simulink model "SIXDOF28"  (R2025b)
settings: Solver=VariableStepAuto  StartTime=0.0  StopTime=sortieStopTime_s  MaxStep=2.0  RelTol=1e-3
undefined symbols (not defined in the file): aircraft_mass, alpha0, alpha_bp, b, CL_table, ClCsurfaces, Cldampingrates, Cldeltae, CmCsurfaces, Cmdampingrates, CnCsurfaces, Cndampingrates, COP, CruiseSpeed, deg, density, DiscIntNeverNeededParam, dwGrad, ElTrim, g, h0, InitialHeadingRadBySortie, InitialPosBySortie, InitPitch, InitUb, Initwb, l, lt, maxPropRad, payloadvolume, PitchTrim, rad, rho, s, S, selectedSortie, St, ThrottleTrim
libraries: slpidlib x12, aerolibasang x3, aerolibconvert2 x2, aerolibadyn x1
(part 2 of 3)

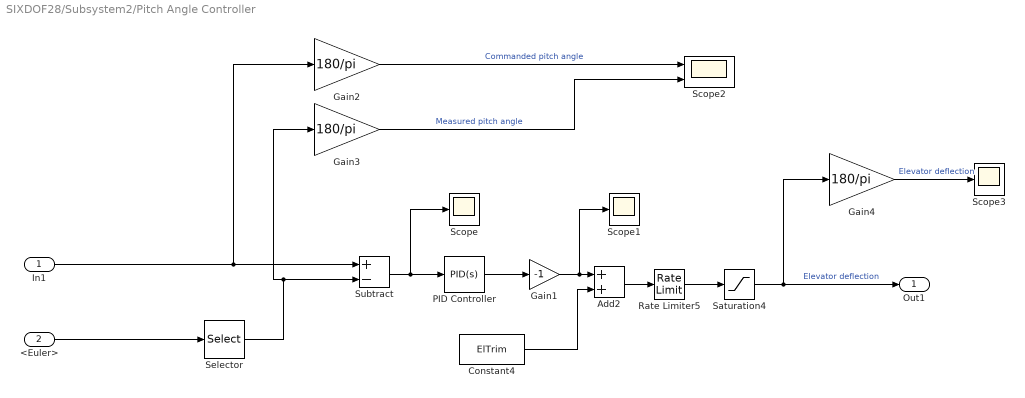
== system SIXDOF28/Subsystem2/Pitch Angle Controller ==
  In1 : Inport
  <Euler> : Inport  Port=2
  Add2 : Sum
  Constant4 : Constant  Value=ElTrim
  Gain1 : Gain  Gain=-1
  Gain2 : Gain  Gain=180/pi
  Gain3 : Gain  Gain=180/pi
  Gain4 : Gain  Gain=180/pi
  PID Controller : slpidlib/PID Controller  Controller=PID  Form=Parallel  TimeDomain=Continuous-time  UseExternalTs=off  SampleTime=-1  IntegratorMethod=Forward Euler  FilterMethod=Forward Euler  ControllerParametersSource=internal  P=1  I=0.2  UseKiTs=off  D=0.1  UseExternalDerivativeSource=off  N=100  UseFilter=on  TunerSelectOption=Transfer Function Based (PID Tuner App)  InitialConditionSource=internal  InitialConditionForIntegrator=0  InitialConditionForFilter=0  DifferentiatorICPrevScaledInput=0  ExternalReset=none  TrackingMode=off  Kt=1  LimitOutput=off  SatLimitsSource=internal  UpperSaturationLimit=inf  LowerSaturationLimit=-inf  LinearizeAsGain=on  AntiWindupMode=none  Kb=1  LimitIntegrator=off  UpperIntegratorSaturationLimit=inf  LowerIntegratorSaturationLimit=-inf  POutMin=[]  POutMax=[]  IOutMin=[]  IOutMax=[]  DOutMin=[]  DOutMax=[]  NOutMin=[]  NOutMax=[]  SumOutMin=[]  SumOutMax=[]  SaturationOutMin=[]  SaturationOutMax=[]  PParamMin=[]  PParamMax=[]  IParamMin=[]  IParamMax=[]  DParamMin=[]  DParamMax=[]  NParamMin=[]  NParamMax=[]  KbParamMin=[]  KbParamMax=[]  KtParamMin=[]  KtParamMax=[]  KbOutMin=[]  KbOutMax=[]  KtOutMin=[]  KtOutMax=[]  IntegratorOutMin=[]  IntegratorOutMax=[]  FilterOutMin=[]  FilterOutMax=[]  SumI1OutMin=[]  SumI1OutMax=[]  SumI2OutMin=[]  SumI2OutMax=[]  SumI3OutMin=[]  SumI3OutMax=[]  SumI4OutMin=[]  SumI4OutMax=[]  SumDOutMin=[]  SumDOutMax=[]  DifferentiatorOutMin=[]  DifferentiatorOutMax=[]  FilterDiffOutCoefMin=[]  FilterDiffOutCoefMax=[]  ReciprocalOutMin=[]  ReciprocalOutMax=[]  SumDenOutMin=[]  SumDenOutMax=[]  SumNumOutMin=[]  SumNumOutMax=[]  DivideOutMin=[]  DivideOutMax=[]  UdiffTsProdOutMin=[]  UdiffTsProdOutMax=[]  NTsProdOutMin=[]  NTsProdOutMax=[]  UintegralTsProdOutMin=[]  UintegralTsProdOutMax=[]  UngainTsProdOutMin=[]  UngainTsProdOutMax=[]  ClampingZeroOutDataTypeStr=Inherit: Inherit via back propagation  ClampingZeroOutMin=[]  ClampingZeroOutMax=[]  FilterDenConstantOutDataTypeStr=Inherit: Inherit via back propagation  FilterDenConstantOutMin=[]  FilterDenConstantOutMax=[]  PCopyOutDataTypeStr=Inherit: Inherit via back propagation  PCopyOutMin=[]  PCopyOutMax=[]  NCopyOutDataTypeStr=Inherit: Inherit via back propagation  NCopyOutMin=[]  NCopyOutMax=[]  IntegratorContinuousStateAttributes=''  IntegratorStateMustResolveToSignalObject=off  IntegratorRTWStateStorageClass=Auto  FilterContinuousStateAttributes=''  FilterStateMustResolveToSignalObject=off  FilterRTWStateStorageClass=Auto  ParallelPVariant=InternalParameters  IdealPVariant=Disabled  IVariant=InternalParameters  DVariant=InternalParameters  IntegratorVariant=Continuous  SatVariant=Disabled  AWVariant=Passthrough  PCopyVariant=Disabled  TRVariant=Disabled  FdbkBlocksVariant=Forward  IdealPFdbkVariant=Disabled  SatFdbkVariant=Disabled  DerivativeFilterVariant=ContFilter  NVariant=InternalParameters  NCopyVariant=Disabled  FilterICVariant=InternalICsFilter  IntegratorICVariant=InternalICs  ExternalResetVariant=Disabled  TRSumVariant=Passthrough  SumFdbkVariant=Disabled  SumVariant=Sum_PID  TsampFilterVariant=InternalTs  TsampNgainVariant=Passthrough  TsampIntegralVariant=Disabled_SignalSpec  ExternalSaturationOutDataTypeStr=Inherit: Same as second input  DerivativeSourceVariant=ErrorSignal  PreIntVariant=InternalPreInt
  Rate Limiter5 : RateLimiter  RisingSlewLimit=1.9  FallingSlewLimit=-1.9
  Saturation4 : Saturate  UpperLimit=21*(pi/180)  LowerLimit=-21*(pi/180)
  Scope : Scope
      settings: ActiveDisplayYMinimum=-1  ActiveDisplayYMaximum=1  DataLoggingVariableName=ScopeData3
  Scope1 : Scope
      settings: ActiveDisplayYMinimum=-1  ActiveDisplayYMaximum=1  DataLoggingVariableName=ScopeData4
  Scope2 : Scope  NumInputPorts=2
      settings: Title=Full Spray mission - Sortie 46  ActiveDisplayYMinimum=-9.9138106361202727  ActiveDisplayYMaximum=18.372173072450739  DataLoggingVariableName=ScopeData56
  Scope3 : Scope
      settings: DataLoggingVariableName=ScopeData81
  Selector : Selector  InputPortWidth=3  IndexOptions=Index vector (dialog)  Indices=[2]  OutputSizes=1
  Subtract : Sum  Inputs=+-
  Out1 : Outport
  wires:
  Gain3/1 -> Scope2/2  "Measured pitch angle"
  Rate Limiter5/1 -> Saturation4/1
  Add2/1 -> Rate Limiter5/1
  Constant4/1 -> Add2/2
  Subtract/1 -> PID Controller/1, Scope/1
  Selector/1 -> Subtract/2, Gain3/1
  In1/1 -> Subtract/1, Gain2/1
  Gain2/1 -> Scope2/1  "Commanded pitch angle"
  PID Controller/1 -> Gain1/1
  <Euler>/1 -> Selector/1
  Gain1/1 -> Scope1/1, Add2/1
  Saturation4/1 -> Gain4/1, Out1/1  "Elevator deflection"
  Gain4/1 -> Scope3/1  "Elevator deflection"

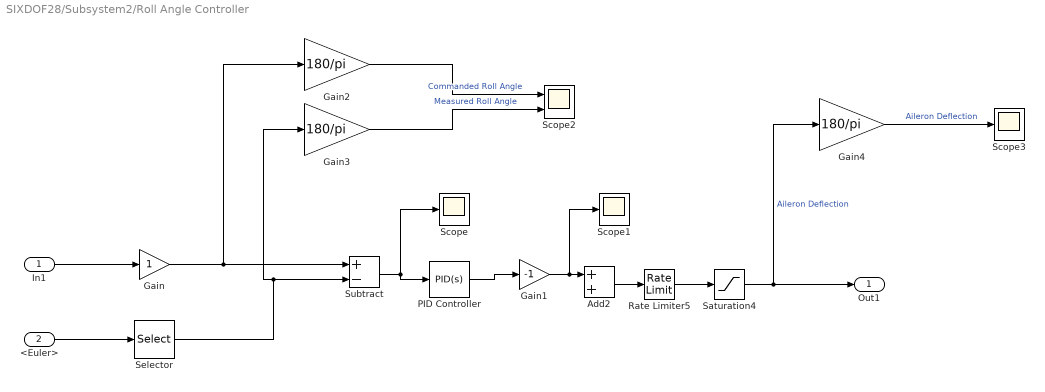
== system SIXDOF28/Subsystem2/Roll Angle Controller ==
  In1 : Inport
  <Euler> : Inport  Port=2
  Add2 : Sum
  Gain : Gain
  Gain1 : Gain  Gain=-1
  Gain2 : Gain  Gain=180/pi
  Gain3 : Gain  Gain=180/pi
  Gain4 : Gain  Gain=180/pi
  PID Controller : slpidlib/PID Controller  Controller=PID  Form=Parallel  TimeDomain=Continuous-time  UseExternalTs=off  SampleTime=-1  IntegratorMethod=Forward Euler  FilterMethod=Forward Euler  ControllerParametersSource=internal  P=5  I=0  UseKiTs=off  D=0  UseExternalDerivativeSource=off  N=100  UseFilter=on  TunerSelectOption=Transfer Function Based (PID Tuner App)  InitialConditionSource=internal  InitialConditionForIntegrator=0  InitialConditionForFilter=0  DifferentiatorICPrevScaledInput=0  ExternalReset=none  TrackingMode=off  Kt=1  LimitOutput=off  SatLimitsSource=internal  UpperSaturationLimit=inf  LowerSaturationLimit=-inf  LinearizeAsGain=on  AntiWindupMode=none  Kb=1  LimitIntegrator=off  UpperIntegratorSaturationLimit=inf  LowerIntegratorSaturationLimit=-inf  POutMin=[]  POutMax=[]  IOutMin=[]  IOutMax=[]  DOutMin=[]  DOutMax=[]  NOutMin=[]  NOutMax=[]  SumOutMin=[]  SumOutMax=[]  SaturationOutMin=[]  SaturationOutMax=[]  PParamMin=[]  PParamMax=[]  IParamMin=[]  IParamMax=[]  DParamMin=[]  DParamMax=[]  NParamMin=[]  NParamMax=[]  KbParamMin=[]  KbParamMax=[]  KtParamMin=[]  KtParamMax=[]  KbOutMin=[]  KbOutMax=[]  KtOutMin=[]  KtOutMax=[]  IntegratorOutMin=[]  IntegratorOutMax=[]  FilterOutMin=[]  FilterOutMax=[]  SumI1OutMin=[]  SumI1OutMax=[]  SumI2OutMin=[]  SumI2OutMax=[]  SumI3OutMin=[]  SumI3OutMax=[]  SumI4OutMin=[]  SumI4OutMax=[]  SumDOutMin=[]  SumDOutMax=[]  DifferentiatorOutMin=[]  DifferentiatorOutMax=[]  FilterDiffOutCoefMin=[]  FilterDiffOutCoefMax=[]  ReciprocalOutMin=[]  ReciprocalOutMax=[]  SumDenOutMin=[]  SumDenOutMax=[]  SumNumOutMin=[]  SumNumOutMax=[]  DivideOutMin=[]  DivideOutMax=[]  UdiffTsProdOutMin=[]  UdiffTsProdOutMax=[]  NTsProdOutMin=[]  NTsProdOutMax=[]  UintegralTsProdOutMin=[]  UintegralTsProdOutMax=[]  UngainTsProdOutMin=[]  UngainTsProdOutMax=[]  ClampingZeroOutDataTypeStr=Inherit: Inherit via back propagation  ClampingZeroOutMin=[]  ClampingZeroOutMax=[]  FilterDenConstantOutDataTypeStr=Inherit: Inherit via back propagation  FilterDenConstantOutMin=[]  FilterDenConstantOutMax=[]  PCopyOutDataTypeStr=Inherit: Inherit via back propagation  PCopyOutMin=[]  PCopyOutMax=[]  NCopyOutDataTypeStr=Inherit: Inherit via back propagation  NCopyOutMin=[]  NCopyOutMax=[]  IntegratorContinuousStateAttributes=''  IntegratorStateMustResolveToSignalObject=off  IntegratorRTWStateStorageClass=Auto  FilterContinuousStateAttributes=''  FilterStateMustResolveToSignalObject=off  FilterRTWStateStorageClass=Auto  ParallelPVariant=InternalParameters  IdealPVariant=Disabled  IVariant=InternalParameters  DVariant=InternalParameters  IntegratorVariant=Continuous  SatVariant=Disabled  AWVariant=Passthrough  PCopyVariant=Disabled  TRVariant=Disabled  FdbkBlocksVariant=Forward  IdealPFdbkVariant=Disabled  SatFdbkVariant=Disabled  DerivativeFilterVariant=ContFilter  NVariant=InternalParameters  NCopyVariant=Disabled  FilterICVariant=InternalICsFilter  IntegratorICVariant=InternalICs  ExternalResetVariant=Disabled  TRSumVariant=Passthrough  SumFdbkVariant=Disabled  SumVariant=Sum_PID  TsampFilterVariant=InternalTs  TsampNgainVariant=Passthrough  TsampIntegralVariant=Disabled_SignalSpec  ExternalSaturationOutDataTypeStr=Inherit: Same as second input  DerivativeSourceVariant=ErrorSignal  PreIntVariant=InternalPreInt
  Rate Limiter5 : RateLimiter  RisingSlewLimit=2.6  FallingSlewLimit=-2.6  SampleTimeMode=inherited
  Saturation4 : Saturate  UpperLimit=14*(pi/180)  LowerLimit=-14*(pi/180)
  Scope : Scope
      settings: ActiveDisplayYMinimum=-1  ActiveDisplayYMaximum=1  DataLoggingVariableName=ScopeData3
  Scope1 : Scope
      settings: ActiveDisplayYMinimum=-1  ActiveDisplayYMaximum=1  DataLoggingVariableName=ScopeData4
  Scope2 : Scope  NumInputPorts=2
      settings: ActiveDisplayYMinimum=-42.530693080397832  ActiveDisplayYMaximum=41.118768188117421  DataLoggingVariableName=ScopeData56
  Scope3 : Scope
      settings: ActiveDisplayYMinimum=-17.5  ActiveDisplayYMaximum=17.5  DataLoggingVariableName=ScopeData70
  Selector : Selector  InputPortWidth=3  IndexOptions=Index vector (dialog)  Indices=[1]  OutputSizes=1
  Subtract : Sum  Inputs=+-
  Out1 : Outport
  wires:
  Saturation4/1 -> Gain4/1, Out1/1  "Aileron Deflection"
  Gain3/1 -> Scope2/2  "Measured Roll Angle"
  Rate Limiter5/1 -> Saturation4/1
  Add2/1 -> Rate Limiter5/1
  Subtract/1 -> PID Controller/1, Scope/1
  Selector/1 -> Subtract/2, Gain3/1
  Gain2/1 -> Scope2/1  "Commanded Roll Angle"
  PID Controller/1 -> Gain1/1
  <Euler>/1 -> Selector/1
  Gain1/1 -> Scope1/1, Add2/1
  Gain/1 -> Subtract/1, Gain2/1
  In1/1 -> Gain/1
  Gain4/1 -> Scope3/1  "Aileron Deflection"

== system SIXDOF28/Subsystem2/Rudder Controller ==
  In1 : Inport
  Constant : Constant  Value=0
  Gain : Gain
  Gain1 : Gain  Gain=180/pi
  Gain2 : Gain  Gain=180/pi
  "Incidence, Sideslip, & Airspeed" : aerolibasang/Incidence, Sideslip, & Airspeed
  PID Controller : slpidlib/PID Controller  Controller=PID  Form=Parallel  TimeDomain=Continuous-time  UseExternalTs=off  SampleTime=-1  IntegratorMethod=Forward Euler  FilterMethod=Forward Euler  ControllerParametersSource=internal  P=1  I=0  UseKiTs=off  D=0  UseExternalDerivativeSource=off  N=100  UseFilter=on  TunerSelectOption=Transfer Function Based (PID Tuner App)  InitialConditionSource=internal  InitialConditionForIntegrator=0  InitialConditionForFilter=0  DifferentiatorICPrevScaledInput=0  ExternalReset=none  TrackingMode=off  Kt=1  LimitOutput=off  SatLimitsSource=internal  UpperSaturationLimit=inf  LowerSaturationLimit=-inf  LinearizeAsGain=on  AntiWindupMode=none  Kb=1  LimitIntegrator=off  UpperIntegratorSaturationLimit=inf  LowerIntegratorSaturationLimit=-inf  POutMin=[]  POutMax=[]  IOutMin=[]  IOutMax=[]  DOutMin=[]  DOutMax=[]  NOutMin=[]  NOutMax=[]  SumOutMin=[]  SumOutMax=[]  SaturationOutMin=[]  SaturationOutMax=[]  PParamMin=[]  PParamMax=[]  IParamMin=[]  IParamMax=[]  DParamMin=[]  DParamMax=[]  NParamMin=[]  NParamMax=[]  KbParamMin=[]  KbParamMax=[]  KtParamMin=[]  KtParamMax=[]  KbOutMin=[]  KbOutMax=[]  KtOutMin=[]  KtOutMax=[]  IntegratorOutMin=[]  IntegratorOutMax=[]  FilterOutMin=[]  FilterOutMax=[]  SumI1OutMin=[]  SumI1OutMax=[]  SumI2OutMin=[]  SumI2OutMax=[]  SumI3OutMin=[]  SumI3OutMax=[]  SumI4OutMin=[]  SumI4OutMax=[]  SumDOutMin=[]  SumDOutMax=[]  DifferentiatorOutMin=[]  DifferentiatorOutMax=[]  FilterDiffOutCoefMin=[]  FilterDiffOutCoefMax=[]  ReciprocalOutMin=[]  ReciprocalOutMax=[]  SumDenOutMin=[]  SumDenOutMax=[]  SumNumOutMin=[]  SumNumOutMax=[]  DivideOutMin=[]  DivideOutMax=[]  UdiffTsProdOutMin=[]  UdiffTsProdOutMax=[]  NTsProdOutMin=[]  NTsProdOutMax=[]  UintegralTsProdOutMin=[]  UintegralTsProdOutMax=[]  UngainTsProdOutMin=[]  UngainTsProdOutMax=[]  ClampingZeroOutDataTypeStr=Inherit: Inherit via back propagation  ClampingZeroOutMin=[]  ClampingZeroOutMax=[]  FilterDenConstantOutDataTypeStr=Inherit: Inherit via back propagation  FilterDenConstantOutMin=[]  FilterDenConstantOutMax=[]  PCopyOutDataTypeStr=Inherit: Inherit via back propagation  PCopyOutMin=[]  PCopyOutMax=[]  NCopyOutDataTypeStr=Inherit: Inherit via back propagation  NCopyOutMin=[]  NCopyOutMax=[]  IntegratorContinuousStateAttributes=''  IntegratorStateMustResolveToSignalObject=off  IntegratorRTWStateStorageClass=Auto  FilterContinuousStateAttributes=''  FilterStateMustResolveToSignalObject=off  FilterRTWStateStorageClass=Auto  ParallelPVariant=InternalParameters  IdealPVariant=Disabled  IVariant=InternalParameters  DVariant=InternalParameters  IntegratorVariant=Continuous  SatVariant=Disabled  AWVariant=Passthrough  PCopyVariant=Disabled  TRVariant=Disabled  FdbkBlocksVariant=Forward  IdealPFdbkVariant=Disabled  SatFdbkVariant=Disabled  DerivativeFilterVariant=ContFilter  NVariant=InternalParameters  NCopyVariant=Disabled  FilterICVariant=InternalICsFilter  IntegratorICVariant=InternalICs  ExternalResetVariant=Disabled  TRSumVariant=Passthrough  SumFdbkVariant=Disabled  SumVariant=Sum_PID  TsampFilterVariant=InternalTs  TsampNgainVariant=Passthrough  TsampIntegralVariant=Disabled_SignalSpec  ExternalSaturationOutDataTypeStr=Inherit: Same as second input  DerivativeSourceVariant=ErrorSignal  PreIntVariant=InternalPreInt
  Rate Limiter : RateLimiter  RisingSlewLimit=1.9  FallingSlewLimit=-1.9  SampleTimeMode=inherited
  Saturation : Saturate  UpperLimit=20*(pi/180)  LowerLimit=-20*(pi/180)
  Scope{,1..3} (4 alike) : Scope
      Scope settings: ActiveDisplayYMinimum=-4.62461388614994  ActiveDisplayYMaximum=5.1253925033808088  YLabel=Sideslip angle (degrees)  DataLoggingVariableName=ScopeData85
      Scope1 settings: ActiveDisplayYMinimum=-0.10105901044913036  ActiveDisplayYMaximum=0.0935182350570406  DataLoggingVariableName=ScopeData86
      Scope2 settings: ActiveDisplayYMinimum=-1  ActiveDisplayYMaximum=1  DataLoggingVariableName=ScopeData87
      Scope3 settings: ActiveDisplayYMinimum=-1  ActiveDisplayYMaximum=1  DataLoggingVariableName=ScopeData88
  Subtract : Sum  Inputs=+-
  Out1 : Outport
  wires:
  In1/1 -> "Incidence, Sideslip, & Airspeed"/1
  "Incidence, Sideslip, & Airspeed"/2 -> Gain2/1, Subtract/2
  Constant/1 -> Subtract/1
  Subtract/1 -> PID Controller/1, Scope1/1
  Rate Limiter/1 -> Saturation/1
  PID Controller/1 -> Gain/1, Scope2/1
  Saturation/1 -> Gain1/1, Out1/1
  Gain/1 -> Rate Limiter/1
  Gain2/1 -> Scope/1  "Sideslip"
  Gain1/1 -> Scope3/1

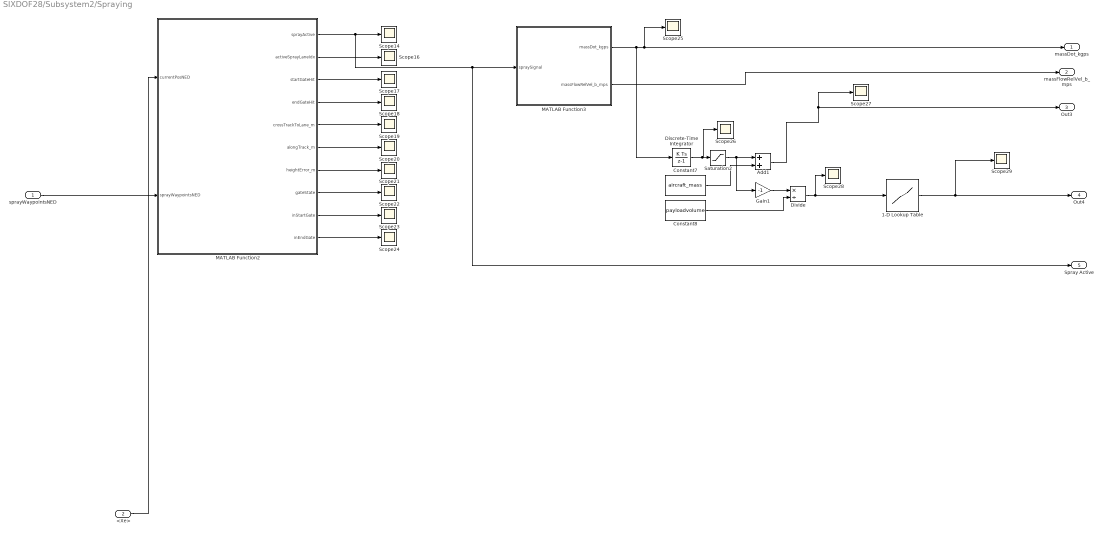
== system SIXDOF28/Subsystem2/Spraying ==
  sprayWaypointsNED : Inport
  <Xe> : Inport  Port=2
  1-D Lookup Table : Lookup_n-D  NumberOfTableDimensions=1  BreakpointsForDimension1=[0 1]  Table=[0.04 0.15]  InternalRulePriority=Speed  RndMeth=Simplest
  Add1 : Sum
  Constant7 : Constant  Value=aircraft_mass
  Constant8 : Constant  Value=payloadvolume
  Discrete-Time Integrator : DiscreteIntegrator  SampleTime=-1  ICPrevOutput=DiscIntNeverNeededParam  ICPrevScaledInput=DiscIntNeverNeededParam
  Divide : Product  Inputs=*/
  Gain1 : Gain  Gain=-1
  MATLAB Function2 : MATLAB Function  TreatAsAtomicUnit=on
  MATLAB Function3 : MATLAB Function  TreatAsAtomicUnit=on
  Saturation2 : Saturate  UpperLimit=0  LowerLimit=-47
  Scope{14,16..29} (15 alike) : Scope
      Scope14 settings: ActiveDisplayYMinimum=-0.12499999999999997  ActiveDisplayYMaximum=1.125  DataLoggingVariableName=ScopeData108
      Scope16 settings: ActiveDisplayYMinimum=0.875  ActiveDisplayYMaximum=2.125  DataLoggingVariableName=ScopeData109
      Scope17 settings: ActiveDisplayYMinimum=-0.12499999999999997  ActiveDisplayYMaximum=1.125  DataLoggingVariableName=ScopeData110
      Scope18 settings: ActiveDisplayYMinimum=-1  ActiveDisplayYMaximum=1  DataLoggingVariableName=ScopeData111
      Scope19 settings: ActiveDisplayYMinimum=-115.21910917677457  ActiveDisplayYMaximum=82.1067049807159  DataLoggingVariableName=ScopeData112
      Scope20 settings: DataLoggingVariableName=ScopeData113
      Scope21 settings: ActiveDisplayYMinimum=-1  ActiveDisplayYMaximum=1  DataLoggingVariableName=ScopeData114
      Scope22 settings: DataLoggingVariableName=ScopeData115
      Scope23 settings: DataLoggingVariableName=ScopeData116
      Scope24 settings: DataLoggingVariableName=ScopeData117
      Scope25 settings: ActiveDisplayYMinimum=-1  ActiveDisplayYMaximum=1  DataLoggingVariableName=ScopeData118
      Scope26 settings: ActiveDisplayYMinimum=-1  ActiveDisplayYMaximum=1  DataLoggingVariableName=ScopeData121
      Scope27 settings: ActiveDisplayYMinimum=-1  ActiveDisplayYMaximum=1  DataLoggingVariableName=ScopeData122
      Scope28 settings: ActiveDisplayYMinimum=-1  ActiveDisplayYMaximum=1  DataLoggingVariableName=ScopeData123
      Scope29 settings: ActiveDisplayYMinimum=-1  ActiveDisplayYMaximum=1  DataLoggingVariableName=ScopeData124
  massDot_kgps : Outport
  massFlowRelVel_b_mps : Outport  Port=2
  Out3 : Outport  Port=3
  Out4 : Outport  Port=4
  Spray Active : Outport  Port=5
  wires:
  MATLAB Function2/5(crossTrackToLane_m) -> Scope19/1
  MATLAB Function2/1(sprayActive) -> Spray Active/1, MATLAB Function3/1(spraySignal), Scope14/1
  MATLAB Function3/1(massDot_kgps) -> Discrete-Time Integrator/1, massDot_kgps/1, Scope25/1
  Add1/1 -> Out3/1, Scope27/1
  MATLAB Function2/9(inStartGate) -> Scope23/1
  Saturation2/1 -> Add1/1, Gain1/1
  MATLAB Function2/4(endGateHit) -> Scope18/1
  MATLAB Function2/6(alongTrack_m) -> Scope20/1
  <Xe>/1 -> MATLAB Function2/1(currentPosNED)
  MATLAB Function2/8(gateState) -> Scope22/1
  Divide/1 -> Scope28/1, 1-D Lookup Table/1
  MATLAB Function2/3(startGateHit) -> Scope17/1
  1-D Lookup Table/1 -> Out4/1, Scope29/1
  Discrete-Time Integrator/1 -> Scope26/1, Saturation2/1
  MATLAB Function2/7(heightError_m) -> Scope21/1
  Constant8/1 -> Divide/2
  Gain1/1 -> Divide/1
  Constant7/1 -> Add1/2
  MATLAB Function2/10(inEndGate) -> Scope24/1
  MATLAB Function2/2(activeSprayLaneIdx) -> Scope16/1
  sprayWaypointsNED/1 -> MATLAB Function2/2(sprayWaypointsNED)
  MATLAB Function3/2(massFlowRelVel_b_mps) -> massFlowRelVel_b_mps/1

== system SIXDOF28/Subsystem2/Throttle Controller ==
  <Vb> : Inport
  Add2 : Sum
  Constant10 : Constant  Value=ThrottleTrim
  Constant9 : Constant  Value=CruiseSpeed
  PID Controller : slpidlib/PID Controller  Controller=PID  Form=Parallel  TimeDomain=Continuous-time  UseExternalTs=off  SampleTime=-1  IntegratorMethod=Forward Euler  FilterMethod=Forward Euler  ControllerParametersSource=internal  P=0.2  I=0.02  UseKiTs=off  D=0  UseExternalDerivativeSource=off  N=100  UseFilter=on  TunerSelectOption=Transfer Function Based (PID Tuner App)  InitialConditionSource=internal  InitialConditionForIntegrator=0  InitialConditionForFilter=0  DifferentiatorICPrevScaledInput=0  ExternalReset=none  TrackingMode=off  Kt=1  LimitOutput=off  SatLimitsSource=internal  UpperSaturationLimit=inf  LowerSaturationLimit=-inf  LinearizeAsGain=on  AntiWindupMode=none  Kb=1  LimitIntegrator=off  UpperIntegratorSaturationLimit=inf  LowerIntegratorSaturationLimit=-inf  POutMin=[]  POutMax=[]  IOutMin=[]  IOutMax=[]  DOutMin=[]  DOutMax=[]  NOutMin=[]  NOutMax=[]  SumOutMin=[]  SumOutMax=[]  SaturationOutMin=[]  SaturationOutMax=[]  PParamMin=[]  PParamMax=[]  IParamMin=[]  IParamMax=[]  DParamMin=[]  DParamMax=[]  NParamMin=[]  NParamMax=[]  KbParamMin=[]  KbParamMax=[]  KtParamMin=[]  KtParamMax=[]  KbOutMin=[]  KbOutMax=[]  KtOutMin=[]  KtOutMax=[]  IntegratorOutMin=[]  IntegratorOutMax=[]  FilterOutMin=[]  FilterOutMax=[]  SumI1OutMin=[]  SumI1OutMax=[]  SumI2OutMin=[]  SumI2OutMax=[]  SumI3OutMin=[]  SumI3OutMax=[]  SumI4OutMin=[]  SumI4OutMax=[]  SumDOutMin=[]  SumDOutMax=[]  DifferentiatorOutMin=[]  DifferentiatorOutMax=[]  FilterDiffOutCoefMin=[]  FilterDiffOutCoefMax=[]  ReciprocalOutMin=[]  ReciprocalOutMax=[]  SumDenOutMin=[]  SumDenOutMax=[]  SumNumOutMin=[]  SumNumOutMax=[]  DivideOutMin=[]  DivideOutMax=[]  UdiffTsProdOutMin=[]  UdiffTsProdOutMax=[]  NTsProdOutMin=[]  NTsProdOutMax=[]  UintegralTsProdOutMin=[]  UintegralTsProdOutMax=[]  UngainTsProdOutMin=[]  UngainTsProdOutMax=[]  ClampingZeroOutDataTypeStr=Inherit: Inherit via back propagation  ClampingZeroOutMin=[]  ClampingZeroOutMax=[]  FilterDenConstantOutDataTypeStr=Inherit: Inherit via back propagation  FilterDenConstantOutMin=[]  FilterDenConstantOutMax=[]  PCopyOutDataTypeStr=Inherit: Inherit via back propagation  PCopyOutMin=[]  PCopyOutMax=[]  NCopyOutDataTypeStr=Inherit: Inherit via back propagation  NCopyOutMin=[]  NCopyOutMax=[]  IntegratorContinuousStateAttributes=''  IntegratorStateMustResolveToSignalObject=off  IntegratorRTWStateStorageClass=Auto  FilterContinuousStateAttributes=''  FilterStateMustResolveToSignalObject=off  FilterRTWStateStorageClass=Auto  ParallelPVariant=InternalParameters  IdealPVariant=Disabled  IVariant=InternalParameters  DVariant=InternalParameters  IntegratorVariant=Continuous  SatVariant=Disabled  AWVariant=Passthrough  PCopyVariant=Disabled  TRVariant=Disabled  FdbkBlocksVariant=Forward  IdealPFdbkVariant=Disabled  SatFdbkVariant=Disabled  DerivativeFilterVariant=ContFilter  NVariant=InternalParameters  NCopyVariant=Disabled  FilterICVariant=InternalICsFilter  IntegratorICVariant=InternalICs  ExternalResetVariant=Disabled  TRSumVariant=Passthrough  SumFdbkVariant=Disabled  SumVariant=Sum_PID  TsampFilterVariant=InternalTs  TsampNgainVariant=Passthrough  TsampIntegralVariant=Disabled_SignalSpec  ExternalSaturationOutDataTypeStr=Inherit: Same as second input  DerivativeSourceVariant=ErrorSignal  PreIntVariant=InternalPreInt
  Saturation1 : Saturate  UpperLimit=1  LowerLimit=0
  Scope{30..34} (5 alike) : Scope
      Scope30 settings: ActiveDisplayYMinimum=-1  ActiveDisplayYMaximum=1  DataLoggingVariableName=ScopeData58
      Scope31 settings: ActiveDisplayYMinimum=-1.5510111091156449  ActiveDisplayYMaximum=1.2326803841963634  DataLoggingVariableName=ScopeData131
      Scope32 settings: ActiveDisplayYMinimum=-1  ActiveDisplayYMaximum=1  DataLoggingVariableName=ScopeData132
      Scope33 settings: ActiveDisplayYMinimum=-1  ActiveDisplayYMaximum=1  DataLoggingVariableName=ScopeData133
      Scope34 settings: ActiveDisplayYMinimum=0.444742326017022  ActiveDisplayYMaximum=1.0517355570110991  DataLoggingVariableName=ScopeData134
  Selector1 : Selector  InputPortWidth=3  IndexOptions=Index vector (dialog)  Indices=[1 ]  OutputSizes=1
  Subtract : Sum  Inputs=+-
  Out1 : Outport
  wires:
  Subtract/1 -> PID Controller/1, Scope31/1
  Constant9/1 -> Subtract/1
  Constant10/1 -> Add2/2
  PID Controller/1 -> Scope32/1, Add2/1
  Saturation1/1 -> Out1/1, Scope34/1
  Add2/1 -> Scope33/1, Saturation1/1
  Selector1/1 -> Scope30/1, Subtract/2
  <Vb>/1 -> Selector1/1

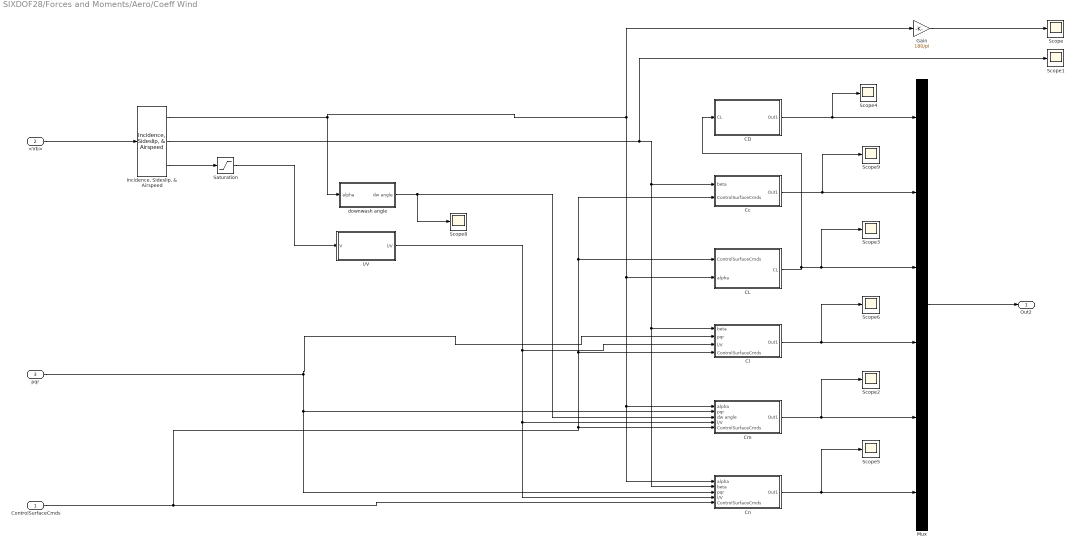
== system SIXDOF28/Forces and Moments/Aero/Coeff Wind ==
  ControlSurfaceCmds : Inport
  <Vb> : Inport  Port=2
  pqr : Inport  Port=3
  CD : Subsystem
  CL : Subsystem
  Cc : Subsystem
  Cl : Subsystem
  Cm : Subsystem
  Cn : Subsystem
  Gain : Gain  Gain=180/pi
  "Incidence, Sideslip, & Airspeed" : aerolibasang/Incidence, Sideslip, & Airspeed
  Mux : Mux  Inputs=6
  Saturation : Saturate  UpperLimit=inf  LowerLimit=0.1
  Scope{,1..6,8..9} (9 alike) : Scope
      Scope settings: ActiveDisplayYMinimum=-205.12693734176204  ActiveDisplayYMaximum=150.84939452113127  DataLoggingVariableName=ScopeData10
      Scope1 settings: ActiveDisplayYMinimum=-0.18233684510886836  ActiveDisplayYMaximum=0.28548639043332236  DataLoggingVariableName=ScopeData11
      Scope2 settings: ActiveDisplayYMinimum=-26.937897847483008  ActiveDisplayYMaximum=2.9998697655158946  DataLoggingVariableName=ScopeData28
      Scope3 settings: ActiveDisplayYMinimum=-1.4592175410693555  ActiveDisplayYMaximum=2.0232265415071504  DataLoggingVariableName=ScopeData6
      Scope4 settings: ActiveDisplayYMinimum=-1  ActiveDisplayYMaximum=1  DataLoggingVariableName=ScopeData7
      Scope5 settings: ActiveDisplayYMinimum=-0.013171688334844891  ActiveDisplayYMaximum=0.013198014472399865  DataLoggingVariableName=ScopeData32
      Scope6 settings: ActiveDisplayYMinimum=-0.01193519980636879  ActiveDisplayYMaximum=0.011614558937549721  DataLoggingVariableName=ScopeData33
      Scope8 settings: ActiveDisplayYMinimum=-1  ActiveDisplayYMaximum=1  DataLoggingVariableName=ScopeData42
      Scope9 settings: ActiveDisplayYMinimum=-1  ActiveDisplayYMaximum=1  DataLoggingVariableName=ScopeData45
  downwash angle : Subsystem
  l/V : Subsystem
  Out2 : Outport
  wires:
  <Vb>/1 -> "Incidence, Sideslip, & Airspeed"/1
  Mux/1 -> Out2/1
  Gain/1 -> Scope/1
  pqr/1 -> Cl/2(pqr), Cn/3(pqr), Cm/2(pqr)
  l/V/1(l/V) -> Cn/4(l/V), Cm/4(l/V), Cl/3(l/V)
  "Incidence, Sideslip, & Airspeed"/3 -> Saturation/1
  downwash angle/1(dw angle) -> Scope8/1, Cm/3(dw angle)
  Cm/1(Out1) -> Mux/5, Scope2/1
  Saturation/1 -> l/V/1(V)
  Cl/1(Out1) -> Mux/4, Scope6/1
  CD/1(Out1) -> Scope4/1, Mux/1
  ControlSurfaceCmds/1 -> Cn/5(ControlSurfaceCmds), Cl/4(ControlSurfaceCmds), CL/1(ControlSurfaceCmds), Cc/2(ControlSurfaceCmds), Cm/5(ControlSurfaceCmds)
  CL/1(CL) -> CD/1(CL), Mux/3, Scope3/1
  "Incidence, Sideslip, & Airspeed"/2 -> Scope1/1, Cn/2(beta), Cl/1(beta), Cc/1(beta)
  Cc/1(Out1) -> Scope9/1, Mux/2
  "Incidence, Sideslip, & Airspeed"/1 -> Gain/1, Cn/1(alpha), Cm/1(alpha), CL/2(alpha), downwash angle/1(alpha)
  Cn/1(Out1) -> Mux/6, Scope5/1

== system SIXDOF28/Forces and Moments/Aero/Coeff Wind/CD ==
  CL : Inport
  Add : Sum
  Constant : Constant  Value=0.45
  Constant2 : Constant  Value=0.07
  Constant3 : Constant  Value=0.13
  Product : Product
  Square : Math  Operator=square
  Subtract : Sum  Inputs=+-
  Out1 : Outport
  wires:
  Product/1 -> Add/1
  Constant3/1 -> Add/2
  Square/1 -> Product/1
  Add/1 -> Out1/1
  CL/1 -> Subtract/1
  Constant/1 -> Subtract/2
  Subtract/1 -> Square/1
  Constant2/1 -> Product/2

== system SIXDOF28/Forces and Moments/Aero/Coeff Wind/CL ==
  ControlSurfaceCmds : Inport
  alpha : Inport  Port=2
  CL wb : Subsystem
  Scope : Scope
      settings: ActiveDisplayYMinimum=0.29326222052096496  ActiveDisplayYMaximum=1.1106400153113154  DataLoggingVariableName=ScopeData53
  Scope1 : Scope
      settings: ActiveDisplayYMinimum=-1  ActiveDisplayYMaximum=1  DataLoggingVariableName=ScopeData128
  Subsystem : Subsystem
  CL : Outport
  wires:
  alpha/1 -> CL wb/1(In1)
  CL wb/1(CL) -> CL/1, Scope/1
  ControlSurfaceCmds/1 -> Subsystem/1(ControlSurfaceCmds)
  Subsystem/1(Out1) -> Scope1/1

== system SIXDOF28/Forces and Moments/Aero/Coeff Wind/Cc ==
  beta : Inport
  ControlSurfaceCmds : Inport  Port=2
  Add : Sum
  Cc beta : Subsystem
  Cc dR : Subsystem
  Scope : Scope
      settings: ActiveDisplayYMinimum=-1  ActiveDisplayYMaximum=1  DataLoggingVariableName=ScopeData49
  Scope1 : Scope
      settings: ActiveDisplayYMinimum=-1  ActiveDisplayYMaximum=1  DataLoggingVariableName=ScopeData16
  Scope2 : Scope
      settings: ActiveDisplayYMinimum=-1  ActiveDisplayYMaximum=1  DataLoggingVariableName=ScopeData61
  Out1 : Outport
  wires:
  Add/1 -> Out1/1, Scope1/1
  beta/1 -> Cc beta/1(In1)
  Cc beta/1(Out1) -> Scope2/1, Add/1
  ControlSurfaceCmds/1 -> Cc dR/1(In1)
  Cc dR/1(Out1) -> Scope/1, Add/2

== system SIXDOF28/Forces and Moments/Aero/Coeff Wind/Cl ==
  beta : Inport
  pqr : Inport  Port=2
  l/V : Inport  Port=3
  ControlSurfaceCmds : Inport  Port=4
  Add : Sum  Inputs=+++
  Cl Csurf : Subsystem
  Cl beta : Subsystem
  Cl pqr : Subsystem
  Scope{,1..4} (5 alike) : Scope
      Scope settings: ActiveDisplayYMinimum=-0.23054850568640728  ActiveDisplayYMaximum=0.23103676274577969  DataLoggingVariableName=ScopeData62
      Scope1 settings: ActiveDisplayYMinimum=-0.24832952525438376  ActiveDisplayYMaximum=0.24682805666661323  DataLoggingVariableName=ScopeData24
      Scope2 settings: ActiveDisplayYMinimum=-1  ActiveDisplayYMaximum=1  DataLoggingVariableName=ScopeData9
      Scope3 settings: DataLoggingVariableName=ScopeData25
      Scope4 settings: ActiveDisplayYMinimum=-0.0026350816975084148  ActiveDisplayYMaximum=0.0050038157278090812  DataLoggingVariableName=ScopeData83
  Sum of Elements : Sum  Inputs=+
  Out1 : Outport
  wires:
  Add/1 -> Sum of Elements/1
  Sum of Elements/1 -> Scope3/1, Out1/1
  beta/1 -> Scope4/1, Cl beta/1(In1)
  Cl beta/1(Out1) -> Scope/1, Add/1
  Cl pqr/1(Out1) -> Scope2/1, Add/2
  pqr/1 -> Cl pqr/1(In1)
  l/V/1 -> Cl pqr/2(In2)
  ControlSurfaceCmds/1 -> Cl Csurf/1(ControlSurfaceCmds)
  Cl Csurf/1(Out1) -> Scope1/1, Add/3

== system SIXDOF28/Forces and Moments/Aero/Coeff Wind/Cm ==
  alpha : Inport
  pqr : Inport  Port=2
  dw angle : Inport  Port=3
  l/V : Inport  Port=4
  ControlSurfaceCmds : Inport  Port=5
  Add1 : Sum  Inputs=+++
  Cm Csurf : Subsystem
  Cm alpha : Subsystem
  Cm pqr : Subsystem
  Scope{,1..3} (4 alike) : Scope
      Scope settings: ActiveDisplayYMinimum=-1  ActiveDisplayYMaximum=1  DataLoggingVariableName=ScopeData35
      Scope1 settings: ActiveDisplayYMinimum=-1  ActiveDisplayYMaximum=1  DataLoggingVariableName=ScopeData53
      Scope2 settings: ActiveDisplayYMinimum=-0.0033252359836460081  ActiveDisplayYMaximum=0.0052138587581284238  DataLoggingVariableName=ScopeData22
      Scope3 settings: ActiveDisplayYMinimum=-1  ActiveDisplayYMaximum=1  DataLoggingVariableName=ScopeData47
  Out1 : Outport
  wires:
  Add1/1 -> Scope3/1, Out1/1
  alpha/1 -> Cm alpha/1(alpha)
  dw angle/1 -> Cm alpha/2(dw angle)
  Cm alpha/1(Out1) -> Scope1/1, Add1/1
  pqr/1 -> Cm pqr/1(In1)
  l/V/1 -> Cm pqr/2(In2)
  Cm pqr/1(Out1) -> Add1/2, Scope2/1
  ControlSurfaceCmds/1 -> Cm Csurf/1(In1)
  Cm Csurf/1(Out1) -> Scope/1, Add1/3

== system SIXDOF28/Forces and Moments/Aero/Coeff Wind/Cn ==
  alpha : Inport
  beta : Inport  Port=2
  pqr : Inport  Port=3
  l/V : Inport  Port=4
  ControlSurfaceCmds : Inport  Port=5
  Add2 : Sum  Inputs=+++
  Cn CSurf : Subsystem
  Cn beta : Subsystem
  Cn pqr : Subsystem
  Scope{,1..3} (4 alike) : Scope
      Scope settings: ActiveDisplayYMinimum=-0.0941958242569857  ActiveDisplayYMaximum=0.094058868274075225  DataLoggingVariableName=ScopeData74
      Scope1 settings: ActiveDisplayYMinimum=-1  ActiveDisplayYMaximum=1  DataLoggingVariableName=ScopeData75
      Scope2 settings: ActiveDisplayYMinimum=-1  ActiveDisplayYMaximum=1  DataLoggingVariableName=ScopeData76
      Scope3 settings: ActiveDisplayYMinimum=-1  ActiveDisplayYMaximum=1  DataLoggingVariableName=ScopeData77
  Sum of Elements3 : Sum  Inputs=+
  Out1 : Outport
  wires:
  Add2/1 -> Sum of Elements3/1
  Sum of Elements3/1 -> Scope3/1, Out1/1
  alpha/1 -> Cn beta/1(In1)
  beta/1 -> Cn beta/2(In2)
  pqr/1 -> Cn pqr/1(In1)
  l/V/1 -> Cn pqr/2(In2)
  Cn pqr/1(Out1) -> Add2/2, Scope1/1
  ControlSurfaceCmds/1 -> Cn CSurf/1(In1)
  Cn CSurf/1(Out1) -> Add2/3, Scope2/1
  Cn beta/1(Out1) -> Scope/1, Add2/1

== system SIXDOF28/Forces and Moments/Aero/Coeff Wind/downwash angle ==
  alpha : Inport
  Constant : Constant  Value=alpha0
  Gain : Gain  Gain=dwGrad
  Subtract : Sum  Inputs=+-
  dw angle : Outport
  wires:
  Constant/1 -> Subtract/2
  alpha/1 -> Subtract/1
  Subtract/1 -> Gain/1
  Gain/1 -> dw angle/1

== system SIXDOF28/Forces and Moments/Aero/Coeff Wind/l//V ==
  V : Inport
  Divide : Product  Inputs=*/
  Saturation : Saturate  UpperLimit=inf  LowerLimit=0
  generalised length : Constant  Value=l
  l/V : Outport
  wires:
  Saturation/1 -> l/V/1  "l/V"
  generalised length/1 -> Divide/1
  Divide/1 -> Saturation/1
  V/1 -> Divide/2

== system SIXDOF28/Forces and Moments/Aero/Coeff Wind/CL/CL wb ==
  In1 : Inport
  1-D Lookup Table1 : Lookup_n-D  NumberOfTableDimensions=1  BreakpointsForDimension1=alpha_bp  Table=CL_table  InternalRulePriority=Speed  RndMeth=Simplest
  Rad to Deg : Gain  Gain=180/pi
  CL : Outport
  wires:
  Rad to Deg/1 -> 1-D Lookup Table1/1
  In1/1 -> Rad to Deg/1
  1-D Lookup Table1/1 -> CL/1

== system SIXDOF28/Forces and Moments/Aero/Coeff Wind/CL/Subsystem ==
  ControlSurfaceCmds : Inport
  Gain : Gain  Gain=Cldeltae
  Scope : Scope
      settings: ActiveDisplayYMinimum=-1  ActiveDisplayYMaximum=1  DataLoggingVariableName=ScopeData129
  Scope1 : Scope
      settings: DataLoggingVariableName=ScopeData130
  Selector : Selector  InputPortWidth=3  IndexOptions=Index vector (dialog)  Indices=[2]  OutputSizes=1
  Out1 : Outport
  wires:
  ControlSurfaceCmds/1 -> Selector/1
  Selector/1 -> Scope/1, Gain/1
  Gain/1 -> Scope1/1, Out1/1

== system SIXDOF28/Forces and Moments/Aero/Coeff Wind/Cc/Cc beta ==
  In1 : Inport
  Gain : Gain  Gain=-1.6
  Out1 : Outport
  wires:
  Gain/1 -> Out1/1
  In1/1 -> Gain/1

== system SIXDOF28/Forces and Moments/Aero/Coeff Wind/Cc/Cc dR ==
  In1 : Inport
  Gain1 : Gain  Gain=0.24
  Scope : Scope
      settings: ActiveDisplayYMinimum=-1  ActiveDisplayYMaximum=1  DataLoggingVariableName=ScopeData15
  Selector : Selector  InputPortWidth=3  IndexOptions=Index vector (dialog)  Indices=[3]  OutputSizes=1
  Out1 : Outport
  wires:
  In1/1 -> Selector/1
  Selector/1 -> Scope/1, Gain1/1
  Gain1/1 -> Out1/1

== system SIXDOF28/Forces and Moments/Aero/Coeff Wind/Cl/Cl Csurf ==
  ControlSurfaceCmds : Inport
  Constant4 : Constant  Value=ClCsurfaces
  Product : Product
  Scope : Scope
      settings: ActiveDisplayYMinimum=-1  ActiveDisplayYMaximum=1  DataLoggingVariableName=ScopeData17
  Scope1 : Scope
      settings: ActiveDisplayYMinimum=-1  ActiveDisplayYMaximum=1  DataLoggingVariableName=ScopeData20
  Scope2 : Scope
      settings: ActiveDisplayYMinimum=-1  ActiveDisplayYMaximum=1  DataLoggingVariableName=ScopeData23
  Sum of Elements1 : Sum  Inputs=+
  Out1 : Outport
  wires:
  ControlSurfaceCmds/1 -> Scope1/1, Product/1
  Constant4/1 -> Scope2/1, Product/2
  Product/1 -> Sum of Elements1/1, Scope/1
  Sum of Elements1/1 -> Out1/1

== system SIXDOF28/Forces and Moments/Aero/Coeff Wind/Cl/Cl beta ==
  In1 : Inport
  Gain : Gain  Gain=-1.4
  Out1 : Outport
  wires:
  Gain/1 -> Out1/1
  In1/1 -> Gain/1

== system SIXDOF28/Forces and Moments/Aero/Coeff Wind/Cl/Cl pqr ==
  In1 : Inport
  In2 : Inport  Port=2
  Constant : Constant  Value=Cldampingrates
  Product : Product
  Product1 : Product
  Scope : Scope
      settings: ActiveDisplayYMinimum=-1  ActiveDisplayYMaximum=1  DataLoggingVariableName=ScopeData5
  Scope1 : Scope
      settings: ActiveDisplayYMinimum=-1  ActiveDisplayYMaximum=1  DataLoggingVariableName=ScopeData8
  Scope3 : Scope
      settings: DataLoggingVariableName=ScopeData59
  Sum of Elements : Sum  Inputs=+
  Out1 : Outport
  wires:
  Constant/1 -> Product1/2
  Product/1 -> Scope1/1, Product1/1
  Product1/1 -> Sum of Elements/1
  In2/1 -> Scope3/1, Product/2
  In1/1 -> Product/1, Scope/1
  Sum of Elements/1 -> Out1/1

== system SIXDOF28/Forces and Moments/Aero/Coeff Wind/Cm/Cm Csurf ==
  In1 : Inport
  Constant4 : Constant  Value=CmCsurfaces
  Product4 : Product
  Scope : Scope
      settings: ActiveDisplayYMinimum=-1  ActiveDisplayYMaximum=1  DataLoggingVariableName=ScopeData48
  Scope1 : Scope
      settings: ActiveDisplayYMinimum=-1  ActiveDisplayYMaximum=1  DataLoggingVariableName=ScopeData63
  Scope10 : Scope
      settings: ActiveDisplayYMinimum=-1  ActiveDisplayYMaximum=1  DataLoggingVariableName=ScopeData50
  Sum of Elements1 : Sum  Inputs=+
  Out1 : Outport
  wires:
  In1/1 -> Scope/1, Product4/1
  Product4/1 -> Sum of Elements1/1, Scope10/1
  Constant4/1 -> Product4/2, Scope1/1
  Sum of Elements1/1 -> Out1/1

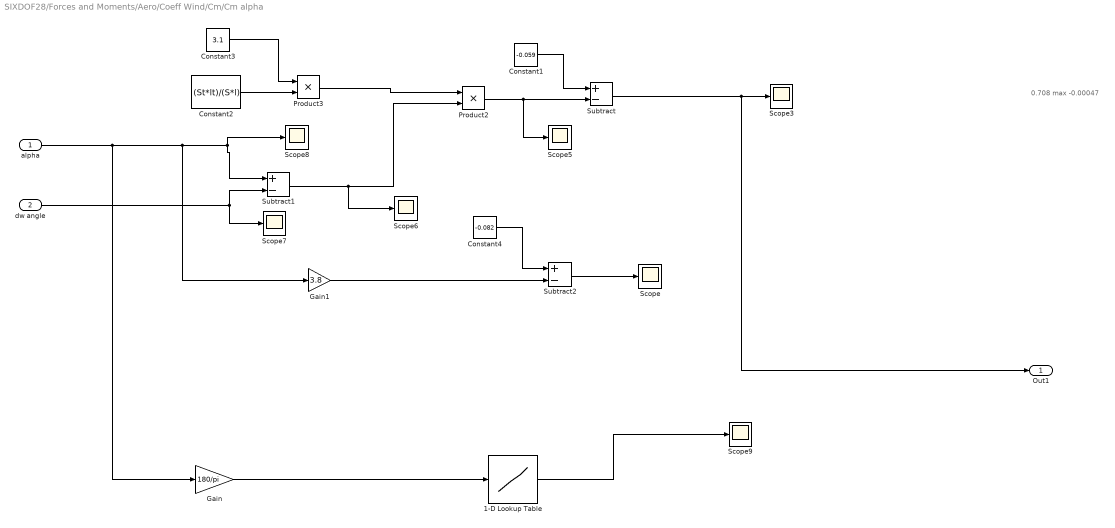
== system SIXDOF28/Forces and Moments/Aero/Coeff Wind/Cm/Cm alpha ==
  note: 0.708 max
      |
      | -0.00047
  alpha : Inport
  dw angle : Inport  Port=2
  1-D Lookup Table : Lookup_n-D  NumberOfTableDimensions=1  BreakpointsForDimension1=[-4 14]  Table=[0.15 -0.15]  InternalRulePriority=Speed  RndMeth=Simplest
  Constant1 : Constant  Value=-0.059
  Constant2 : Constant  Value=(St*lt)/(S*l)
  Constant3 : Constant  Value=3.1
  Constant4 : Constant  Value=-0.082
  Gain : Gain  Gain=180/pi
  Gain1 : Gain  Gain=3.8
  Product2 : Product
  Product3 : Product
  Scope{,3,5..9} (7 alike) : Scope
      Scope settings: ActiveDisplayYMinimum=-0.47069996615447218  ActiveDisplayYMaximum=-0.038811114871725325  DataLoggingVariableName=ScopeData67
      Scope3 settings: ActiveDisplayYMinimum=-0.43175351545914425  ActiveDisplayYMaximum=0.062572502115878989  DataLoggingVariableName=ScopeData34
      Scope5 settings: ActiveDisplayYMinimum=-1  ActiveDisplayYMaximum=1  DataLoggingVariableName=ScopeData36
      Scope6 settings: ActiveDisplayYMinimum=-1  ActiveDisplayYMaximum=1  DataLoggingVariableName=ScopeData37
      Scope7 settings: ActiveDisplayYMinimum=-1  ActiveDisplayYMaximum=1  DataLoggingVariableName=ScopeData38
      Scope8 settings: ActiveDisplayYMinimum=-1  ActiveDisplayYMaximum=1  DataLoggingVariableName=ScopeData39
      Scope9 settings: ActiveDisplayYMinimum=0.068678805629467779  ActiveDisplayYMaximum=0.07207909787052813  DataLoggingVariableName=ScopeData64
  Subtract : Sum  Inputs=+-
  Subtract1 : Sum  Inputs=+-
  Subtract2 : Sum  Inputs=+-
  Out1 : Outport
  wires:
  Constant3/1 -> Product3/1
  dw angle/1 -> Scope7/1, Subtract1/2
  Product2/1 -> Scope5/1, Subtract/2
  Subtract1/1 -> Scope6/1, Product2/2
  Subtract/1 -> Out1/1, Scope3/1
  Constant2/1 -> Product3/2
  alpha/1 -> Gain/1, Gain1/1, Subtract1/1, Scope8/1
  Product3/1 -> Product2/1
  Gain/1 -> 1-D Lookup Table/1
  1-D Lookup Table/1 -> Scope9/1
  Gain1/1 -> Subtract2/2
  Constant4/1 -> Subtract2/1
  Subtract2/1 -> Scope/1
  Constant1/1 -> Subtract/1

== system SIXDOF28/Forces and Moments/Aero/Coeff Wind/Cm/Cm pqr ==
  In1 : Inport
  In2 : Inport  Port=2
  Constant : Constant  Value=Cmdampingrates
  Product : Product
  Product1 : Product
  Scope : Scope
      settings: ActiveDisplayYMinimum=-1  ActiveDisplayYMaximum=1  DataLoggingVariableName=ScopeData12
  Scope1 : Scope
      settings: ActiveDisplayYMinimum=-1  ActiveDisplayYMaximum=1  DataLoggingVariableName=ScopeData21
  Sum of Elements : Sum  Inputs=+
  Out1 : Outport
  wires:
  In1/1 -> Product/1, Scope/1
  Product1/1 -> Sum of Elements/1
  Constant/1 -> Product1/2
  In2/1 -> Product/2
  Product/1 -> Scope1/1, Product1/1
  Sum of Elements/1 -> Out1/1

== system SIXDOF28/Forces and Moments/Aero/Coeff Wind/Cn/Cn CSurf ==
  In1 : Inport
  Constant2 : Constant  Value=CnCsurfaces
  Product3 : Product
  Scope7 : Scope
      settings: ActiveDisplayYMinimum=-1  ActiveDisplayYMaximum=1  DataLoggingVariableName=ScopeData55
  Sum of Elements2 : Sum  Inputs=+
  Out1 : Outport
  wires:
  Product3/1 -> Sum of Elements2/1, Scope7/1
  Constant2/1 -> Product3/2
  Sum of Elements2/1 -> Out1/1
  In1/1 -> Product3/1

== system SIXDOF28/Forces and Moments/Aero/Coeff Wind/Cn/Cn beta ==
  In1 : Inport
  In2 : Inport  Port=2
  Constant1 : Constant
  Gain : Gain  Gain=180/(15*pi)
  Product2 : Product
  Scope : Scope
      settings: ActiveDisplayYMinimum=-1  ActiveDisplayYMaximum=1  DataLoggingVariableName=ScopeData78
  Scope4 : Scope
      settings: ActiveDisplayYMinimum=-1  ActiveDisplayYMaximum=1  DataLoggingVariableName=ScopeData46
  Subtract : Sum  Inputs=+-
  Out1 : Outport
  wires:
  In1/1 -> Gain/1
  Subtract/1 -> Product2/1
  Gain/1 -> Subtract/2
  In2/1 -> Product2/2, Scope4/1
  Constant1/1 -> Subtract/1
  Product2/1 -> Scope/1, Out1/1

== system SIXDOF28/Forces and Moments/Aero/Coeff Wind/Cn/Cn pqr ==
  In1 : Inport
  In2 : Inport  Port=2
  Constant : Constant  Value=Cndampingrates
  Product : Product
  Product1 : Product
  Scope{,1..3} (4 alike) : Scope
      Scope settings: ActiveDisplayYMinimum=-0.12499999999999997  ActiveDisplayYMaximum=1.125  DataLoggingVariableName=ScopeData29
      Scope1 settings: ActiveDisplayYMinimum=-1  ActiveDisplayYMaximum=1  DataLoggingVariableName=ScopeData30
      Scope2 settings: ActiveDisplayYMinimum=-1  ActiveDisplayYMaximum=1  DataLoggingVariableName=ScopeData31
      Scope3 settings: ActiveDisplayYMinimum=-1  ActiveDisplayYMaximum=1  DataLoggingVariableName=ScopeData79
  Sum of Elements : Sum  Inputs=+
  Out1 : Outport
  wires:
  In1/1 -> Product/1, Scope/1
  Constant/1 -> Product1/2
  Product/1 -> Scope1/1, Product1/1
  In2/1 -> Product/2
  Product1/1 -> Sum of Elements/1, Scope2/1
  Sum of Elements/1 -> Scope3/1, Out1/1

== matlab function SIXDOF28/Subsystem2/Flight Controller/MATLAB Function1 ==
  data: vehiclePosNED input; crossTrackError_m output; vehicleVelNED input; waypointsNED input; crossTrackRate_mps output; alongTrackRate_mps output; activeLegIdxIn input; waypointRadius_m input; activeLegIdxOut output; switchFlag output; distanceToWaypointB_m output; closestPointNED output; altitudeCmd_m output
function [crossTrackError_m, crossTrackRate_mps, alongTrackRate_mps, ...
    activeLegIdxOut, switchFlag, distanceToWaypointB_m, closestPointNED, ...
    altitudeCmd_m] = ...
    crossTrackErrorABNED(vehiclePosNED, vehicleVelNED, waypointsNED, ...
    activeLegIdxIn, waypointRadius_m)
%#codegen
% crossTrackErrorABNED
% Simulink-friendly cross-track calculation with ArduPilot-style mission
% leg advance logic for a waypoint list in NED coordinates.
%
% Inputs:
%   vehiclePosNED   [1x3] or [3x1] current position [North East Down] [m]
%   vehicleVelNED   [1x3] or [3x1] current velocity [North East Down] [m/s]
%   waypointsNED    [Nx3] waypoint matrix [North East Down] [m]
%   activeLegIdxIn  active leg index. Leg i uses rows i and i+1.
%   waypointRadius_m mission waypoint radius used for leg switching [m]
%
% Outputs:
%   crossTrackError_m     signed horizontal cross-track error [m]
%   crossTrackRate_mps    signed horizontal cross-track rate [m/s]
%   alongTrackRate_mps    along-track rate [m/s]
%   activeLegIdxOut       updated active leg index after switch logic
%   switchFlag            1 when a leg switch occurred this call, else 0
%   distanceToWaypointB_m horizontal distance to the current waypoint B [m]
%   closestPointNED       closest point on the active waypoint leg [N E D]
%   altitudeCmd_m         desired altitude [m], positive Up
%
% Notes:
% - This matches the ArduPilot-style horizontal calculation on the active
%   waypoint leg using the N/E components only.
% - altitudeCmd_m follows purePursuitGuidanceNED and commands the altitude
%   of the next active waypoint directly.
% - Sign convention follows the 2D scalar cross product:
%       u %% v = u_N*v_E - u_E*v_N
% - Mission leg advance occurs when either:
%       1) distance to waypoint B <= waypointRadius_m, or
%       2) the aircraft crosses the finish line at waypoint B, defined as
%          the line through B perpendicular to the inbound leg A->B

    pos = zeros(1,3);
    vel = zeros(1,3);
    pos(1) = vehiclePosNED(1);
    pos(2) = vehiclePosNED(2);
    pos(3) = vehiclePosNED(3);
    vel(1) = vehicleVelNED(1);
    vel(2) = vehicleVelNED(2);
    vel(3) = vehicleVelNED(3);

    crossTrackError_m = 0.0;
    crossTrackRate_mps = 0.0;
    alongTrackRate_mps = 0.0;
    activeLegIdxOut = 1;
    switchFlag = 0.0;
    distanceToWaypointB_m = 0.0;
    closestPointNED = pos;
    altitudeCmd_m = -pos(3);
    switchReasonCode = 0.0;

    waypointCount = size(waypointsNED, 1);
    if waypointCount < 2 || size(waypointsNED, 2) < 3
        if waypointCount == 1 && size(waypointsNED, 2) >= 3
            altitudeCmd_m = -waypointsNED(1,3);
        end
        return
    end

    if ~isfinite(activeLegIdxIn)
        activeLegIdxIn = 1;
    end
    activeLegIdxOut = floor(activeLegIdxIn);
    activeLegIdxOut = min(max(activeLegIdxOut, 1), waypointCount - 1);

    if ~isfinite(waypointRadius_m) || waypointRadius_m < 0.0
        waypointRadius_m = 0.0;
    end

    while activeLegIdxOut < waypointCount
        wpA = waypointsNED(activeLegIdxOut, :);
        wpB = waypointsNED(activeLegIdxOut + 1, :);
        AB_NE = [wpB(1) - wpA(1), wpB(2) - wpA(2)];
        AB_norm = hypot(AB_NE(1), AB_NE(2));

        if AB_norm <= 1e-9
            if activeLegIdxOut < waypointCount - 1
                activeLegIdxOut = activeLegIdxOut + 1;
                switchReasonCode = 3.0;
                continue
            else
                closestPointNED = wpB;
                altitudeCmd_m = -wpB(3);
                switchFlag = double(switchReasonCode ~= 0.0);
                return
            end
        end

        distanceToWaypointB_m = hypot(pos(1) - wpB(1), pos(2) - wpB(2));
        finishLineCrossed = ((pos(1) - wpB(1)) * AB_NE(1) + ...
            (pos(2) - wpB(2)) * AB_NE(2)) >= 0.0;

        if activeLegIdxOut < waypointCount - 1 && distanceToWaypointB_m <= waypointRadius_m
            activeLegIdxOut = activeLegIdxOut + 1;
            switchReasonCode = 1.0;
            continue
        end

        if activeLegIdxOut < waypointCount - 1 && finishLineCrossed
            activeLegIdxOut = activeLegIdxOut + 1;
            switchReasonCode = 2.0;
            continue
        end

        break
    end

    wpA = waypointsNED(activeLegIdxOut, :);
    wpB = waypointsNED(activeLegIdxOut + 1, :);
    AB_NE = [wpB(1) - wpA(1), wpB(2) - wpA(2)];
    AB_norm = hypot(AB_NE(1), AB_NE(2));

    if AB_norm <= 1e-9
        closestPointNED = wpB;
        distanceToWaypointB_m = hypot(pos(1) - wpB(1), pos(2) - wpB(2));
        altitudeCmd_m = -wpB(3);
        switchFlag = double(switchReasonCode ~= 0.0);
        return
    end

    AB_unit = AB_NE / AB_norm;
    A_air_NE = [pos(1) - wpA(1), pos(2) - wpA(2)];
    vel_NE = [vel(1), vel(2)];
    sStarRaw = (A_air_NE(1) * AB_NE(1) + A_air_NE(2) * AB_NE(2)) / (AB_norm^2);
    sStarClamped = min(max(sStarRaw, 0.0), 1.0);

    closestPointNED = wpA + sStarClamped * (wpB - wpA);
    distanceToWaypointB_m = hypot(pos(1) - wpB(1), pos(2) - wpB(2));

    crossTrackError_m = A_air_NE(1) * AB_unit(2) - A_air_NE(2) * AB_unit(1);
    crossTrackRate_mps = vel_NE(1) * AB_unit(2) - vel_NE(2) * AB_unit(1);
    alongTrackRate_mps = vel_NE(1) * AB_unit(1) + vel_NE(2) * AB_unit(2);
    altitudeCmd_m = -wpB(3);
    switchFlag = double(switchReasonCode ~= 0.0);
end
